simulink library "mobileRoboticsLib"  (R2022b)
settings: Solver=VariableStepAuto  StartTime=0.0  StopTime=10.0  RelTol=1e-3
undefined symbols (not defined in the file or in its folder): DiscIntNeverNeededParam, X, Y, Z
libraries: sm_lib x67, nesl_utility x25, $bdroot x12
(part 4 of 4)

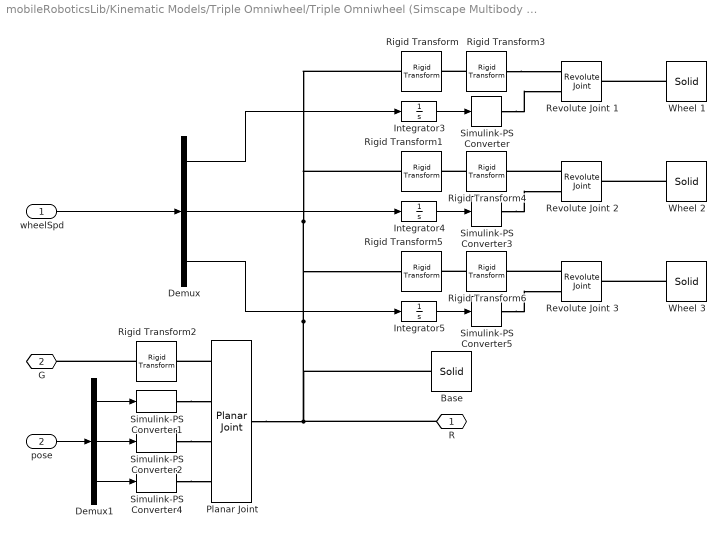
== system mobileRoboticsLib/Kinematic Models/Triple Omniwheel/Triple Omniwheel (Simscape Multibody Model) ==
  wheelSpd : Inport
  pose : Inport  Port=2
  Base : sm_lib/Body Elements/Solid  GraphicAmbientColor=[0.15 0.15 0.15 1.0]  BasedOnType=Mass  CenterOfMass=[0 0 0]  CenterOfMassUnits=m  GraphicDiffuseColor=chassisColor  CylinderLength=chassisThickness  CylinderLengthUnits=m  CylinderRadius=robotRadius-(wheelThickness/2)  CylinderRadiusUnits=m  Density=chassisMass  DensityUnits=kg/m^3  DoExposeReferenceFrame=on  GraphicEmissiveColor=[0.0 0.0 0.0 1.0]  ExportEntireGeometry=off  SerializedFrames=<Frames/>  MarkerShape=Sphere  MarkerSize=10  GraphicType=FromGeometry  InertiaType=CalculateFromGeometry  Mass=chassisMass  MassUnits=kg  MomentsOfInertia=[1 1 1]  MomentsOfInertiaUnits=kg*m^2  GraphicOpacity=1.0  ProductsOfInertia=[1 1 1]  ProductsOfInertiaUnits=kg*m^2  GraphicShininess=75  GraphicSpecularColor=[0.5 0.5 0.5 1.0]  GraphicVisPropType=SimpleVisualProperties  GeometryShape=Cylinder
  Demux : Demux  Outputs=3
  Demux1 : Demux  Outputs=3
  Integrator3 : Integrator
  Integrator4 : Integrator
  Integrator5 : Integrator
  Planar Joint : sm_lib/Joints/Planar Joint  JointMode=Normal  SenseConstraintForce=off  SenseConstraintForceX=off  SenseConstraintForceY=off  SenseConstraintForceZ=off  SenseConstraintTorque=off  SenseConstraintTorqueX=off  SenseConstraintTorqueY=off  SenseConstraintTorqueZ=off  SenseTotalForce=off  SenseTotalForceX=off  SenseTotalForceY=off  SenseTotalForceZ=off  SenseTotalTorque=off  SenseTotalTorqueX=off  SenseTotalTorqueY=off  SenseTotalTorqueZ=off  CompositeWrenchDir=FollowerOnBase  CompositeWrenchFrame=BaseFrame  PxEquilibriumPosition=0  PxEquilibriumPositionUnits=m  PxSpringStiffness=0  PxSpringStiffnessUnits=N/m  PxDampingCoefficient=0  PxDampingCoefficientUnits=N/(m/s)  PxTorqueActuationMode=ComputedTorque  PxMotionActuationMode=InputMotion  PxSensePosition=off  PxSenseVelocity=off  PxSenseAcceleration=off  PxSenseTorqueForce=off  PxSenseLowerLimitTorqueForce=off  PxSenseUpperLimitTorqueForce=off  PxLowerLimitSpecify=off  PxLowerLimitBound=-1  PxLowerLimitBoundUnits=m  PxLowerLimitStiffness=1e6  PxLowerLimitStiffnessUnits=N/m  PxLowerLimitDamping=1e3  PxLowerLimitDampingUnits=N/(m/s)  PxLowerLimitTransitionRegionWidth=1e-4  PxLowerLimitTransitionRegionWidthUnits=m  PxUpperLimitSpecify=off  PxUpperLimitBound=1  PxUpperLimitBoundUnits=m  PxUpperLimitStiffness=1e6  PxUpperLimitStiffnessUnits=N/m  PxUpperLimitDamping=1e3  PxUpperLimitDampingUnits=N/(m/s)  PxUpperLimitTransitionRegionWidth=1e-4  PxUpperLimitTransitionRegionWidthUnits=m  PxPositionTargetSpecify=on  PxPositionTargetPriority=High  PxPositionTargetValue=initX  PxPositionTargetValueUnits=m  PxVelocityTargetSpecify=off  PxVelocityTargetPriority=High  PxVelocityTargetValue=0  PxVelocityTargetValueUnits=m/s  PyEquilibriumPosition=0  PyEquilibriumPositionUnits=m  PySpringStiffness=0  PySpringStiffnessUnits=N/m  PyDampingCoefficient=0  PyDampingCoefficientUnits=N/(m/s)  PyTorqueActuationMode=ComputedTorque  PyMotionActuationMode=InputMotion  PySensePosition=off  PySenseVelocity=off  PySenseAcceleration=off  PySenseTorqueForce=off  PySenseLowerLimitTorqueForce=off  PySenseUpperLimitTorqueForce=off  PyLowerLimitSpecify=off  PyLowerLimitBound=-1  PyLowerLimitBoundUnits=m  PyLowerLimitStiffness=1e6  PyLowerLimitStiffnessUnits=N/m  PyLowerLimitDamping=1e3  PyLowerLimitDampingUnits=N/(m/s)  PyLowerLimitTransitionRegionWidth=1e-4  PyLowerLimitTransitionRegionWidthUnits=m  PyUpperLimitSpecify=off  PyUpperLimitBound=1  PyUpperLimitBoundUnits=m  PyUpperLimitStiffness=1e6  PyUpperLimitStiffnessUnits=N/m  PyUpperLimitDamping=1e3  PyUpperLimitDampingUnits=N/(m/s)  PyUpperLimitTransitionRegionWidth=1e-4  PyUpperLimitTransitionRegionWidthUnits=m  PyPositionTargetSpecify=on  PyPositionTargetPriority=High  PyPositionTargetValue=initY  PyPositionTargetValueUnits=m  PyVelocityTargetSpecify=off  PyVelocityTargetPriority=High  PyVelocityTargetValue=0  PyVelocityTargetValueUnits=m/s  RzEquilibriumPosition=0  RzEquilibriumPositionUnits=deg  RzSpringStiffness=0  RzSpringStiffnessUnits=N*m/deg  RzDampingCoefficient=0  RzDampingCoefficientUnits=N*m/(deg/s)  RzTorqueActuationMode=ComputedTorque  RzMotionActuationMode=InputMotion  RzSensePosition=off  RzSenseVelocity=off  RzSenseAcceleration=off  RzSenseTorqueForce=off  RzSenseLowerLimitTorqueForce=off  RzSenseUpperLimitTorqueForce=off  RzLowerLimitSpecify=off  RzLowerLimitBound=-90  RzLowerLimitBoundUnits=deg  RzLowerLimitStiffness=1e4  RzLowerLimitStiffnessUnits=N*m/deg  RzLowerLimitDamping=10  RzLowerLimitDampingUnits=N*m/(deg/s)  RzLowerLimitTransitionRegionWidth=0.1  RzLowerLimitTransitionRegionWidthUnits=deg  RzUpperLimitSpecify=off  RzUpperLimitBound=90  RzUpperLimitBoundUnits=deg  RzUpperLimitStiffness=1e4  RzUpperLimitStiffnessUnits=N*m/deg  RzUpperLimitDamping=10  RzUpperLimitDampingUnits=N*m/(deg/s)  RzUpperLimitTransitionRegionWidth=0.1  RzUpperLimitTransitionRegionWidthUnits=deg  RzPositionTargetSpecify=on  RzPositionTargetPriority=High  RzPositionTargetValue=initAngle  RzPositionTargetValueUnits=rad  RzVelocityTargetSpecify=off  RzVelocityTargetPriority=High  RzVelocityTargetValue=0  RzVelocityTargetValueUnits=deg/s
  Revolute Joint 1 : sm_lib/Joints/Revolute Joint  JointMode=Normal  SenseConstraintForce=off  SenseConstraintForceX=off  SenseConstraintForceY=off  SenseConstraintForceZ=off  SenseConstraintTorque=off  SenseConstraintTorqueX=off  SenseConstraintTorqueY=off  SenseConstraintTorqueZ=off  SenseTotalForce=off  SenseTotalForceX=off  SenseTotalForceY=off  SenseTotalForceZ=off  SenseTotalTorque=off  SenseTotalTorqueX=off  SenseTotalTorqueY=off  SenseTotalTorqueZ=off  CompositeWrenchDir=FollowerOnBase  CompositeWrenchFrame=BaseFrame  EquilibriumPosition=0  EquilibriumPositionUnits=deg  SpringStiffness=0  SpringStiffnessUnits=N*m/deg  DampingCoefficient=0  DampingCoefficientUnits=N*m/(deg/s)  TorqueActuationMode=ComputedTorque  MotionActuationMode=InputMotion  SensePosition=off  SenseVelocity=off  SenseAcceleration=off  SenseTorqueForce=off  SenseLowerLimitTorqueForce=off  SenseUpperLimitTorqueForce=off  LowerLimitSpecify=off  LowerLimitBound=-90  LowerLimitBoundUnits=deg  LowerLimitStiffness=1e4  LowerLimitStiffnessUnits=N*m/deg  LowerLimitDamping=10  LowerLimitDampingUnits=N*m/(deg/s)  LowerLimitTransitionRegionWidth=0.1  LowerLimitTransitionRegionWidthUnits=deg  UpperLimitSpecify=off  UpperLimitBound=90  UpperLimitBoundUnits=deg  UpperLimitStiffness=1e4  UpperLimitStiffnessUnits=N*m/deg  UpperLimitDamping=10  UpperLimitDampingUnits=N*m/(deg/s)  UpperLimitTransitionRegionWidth=0.1  UpperLimitTransitionRegionWidthUnits=deg  PositionTargetSpecify=off  PositionTargetPriority=High  PositionTargetValue=0  PositionTargetValueUnits=deg  VelocityTargetSpecify=off  VelocityTargetPriority=High  VelocityTargetValue=0  VelocityTargetValueUnits=deg/s
  Revolute Joint 2 : sm_lib/Joints/Revolute Joint  JointMode=Normal  SenseConstraintForce=off  SenseConstraintForceX=off  SenseConstraintForceY=off  SenseConstraintForceZ=off  SenseConstraintTorque=off  SenseConstraintTorqueX=off  SenseConstraintTorqueY=off  SenseConstraintTorqueZ=off  SenseTotalForce=off  SenseTotalForceX=off  SenseTotalForceY=off  SenseTotalForceZ=off  SenseTotalTorque=off  SenseTotalTorqueX=off  SenseTotalTorqueY=off  SenseTotalTorqueZ=off  CompositeWrenchDir=FollowerOnBase  CompositeWrenchFrame=BaseFrame  EquilibriumPosition=0  EquilibriumPositionUnits=deg  SpringStiffness=0  SpringStiffnessUnits=N*m/deg  DampingCoefficient=0  DampingCoefficientUnits=N*m/(deg/s)  TorqueActuationMode=ComputedTorque  MotionActuationMode=InputMotion  SensePosition=off  SenseVelocity=off  SenseAcceleration=off  SenseTorqueForce=off  SenseLowerLimitTorqueForce=off  SenseUpperLimitTorqueForce=off  LowerLimitSpecify=off  LowerLimitBound=-90  LowerLimitBoundUnits=deg  LowerLimitStiffness=1e4  LowerLimitStiffnessUnits=N*m/deg  LowerLimitDamping=10  LowerLimitDampingUnits=N*m/(deg/s)  LowerLimitTransitionRegionWidth=0.1  LowerLimitTransitionRegionWidthUnits=deg  UpperLimitSpecify=off  UpperLimitBound=90  UpperLimitBoundUnits=deg  UpperLimitStiffness=1e4  UpperLimitStiffnessUnits=N*m/deg  UpperLimitDamping=10  UpperLimitDampingUnits=N*m/(deg/s)  UpperLimitTransitionRegionWidth=0.1  UpperLimitTransitionRegionWidthUnits=deg  PositionTargetSpecify=off  PositionTargetPriority=High  PositionTargetValue=0  PositionTargetValueUnits=deg  VelocityTargetSpecify=off  VelocityTargetPriority=High  VelocityTargetValue=0  VelocityTargetValueUnits=deg/s
  Revolute Joint 3 : sm_lib/Joints/Revolute Joint  JointMode=Normal  SenseConstraintForce=off  SenseConstraintForceX=off  SenseConstraintForceY=off  SenseConstraintForceZ=off  SenseConstraintTorque=off  SenseConstraintTorqueX=off  SenseConstraintTorqueY=off  SenseConstraintTorqueZ=off  SenseTotalForce=off  SenseTotalForceX=off  SenseTotalForceY=off  SenseTotalForceZ=off  SenseTotalTorque=off  SenseTotalTorqueX=off  SenseTotalTorqueY=off  SenseTotalTorqueZ=off  CompositeWrenchDir=FollowerOnBase  CompositeWrenchFrame=BaseFrame  EquilibriumPosition=0  EquilibriumPositionUnits=deg  SpringStiffness=0  SpringStiffnessUnits=N*m/deg  DampingCoefficient=0  DampingCoefficientUnits=N*m/(deg/s)  TorqueActuationMode=ComputedTorque  MotionActuationMode=InputMotion  SensePosition=off  SenseVelocity=off  SenseAcceleration=off  SenseTorqueForce=off  SenseLowerLimitTorqueForce=off  SenseUpperLimitTorqueForce=off  LowerLimitSpecify=off  LowerLimitBound=-90  LowerLimitBoundUnits=deg  LowerLimitStiffness=1e4  LowerLimitStiffnessUnits=N*m/deg  LowerLimitDamping=10  LowerLimitDampingUnits=N*m/(deg/s)  LowerLimitTransitionRegionWidth=0.1  LowerLimitTransitionRegionWidthUnits=deg  UpperLimitSpecify=off  UpperLimitBound=90  UpperLimitBoundUnits=deg  UpperLimitStiffness=1e4  UpperLimitStiffnessUnits=N*m/deg  UpperLimitDamping=10  UpperLimitDampingUnits=N*m/(deg/s)  UpperLimitTransitionRegionWidth=0.1  UpperLimitTransitionRegionWidthUnits=deg  PositionTargetSpecify=off  PositionTargetPriority=High  PositionTargetValue=0  PositionTargetValueUnits=deg  VelocityTargetSpecify=off  VelocityTargetPriority=High  VelocityTargetValue=0  VelocityTargetValueUnits=deg/s
  Rigid Transform : sm_lib/Frames and Transforms/Rigid Transform  TranslationMethod=Cartesian  TranslationStandardOffset=0  TranslationLengthUnit=m  TranslationStandardAxis=+Y  TranslationCartesianOffset=[robotRadius*cos(wheelAngles(1)) robotRadius*sin(wheelAngles(1)) 0]  TranslationROffset=0  TranslationROffsetUnits=m  TranslationZOffset=0  TranslationZOffsetUnits=m  TranslationThetaOffset=0  TranslationThetaOffsetUnits=deg  RotationMethod=AlignedAxes  RotationAngleUnits=deg  RotationStandardAxis=+Z  RotationAngle=0.0  RotationArbitraryAxis=[0 0 1]  FollAlignAxisA=+Z  BaseAlignAxisA=+Y  FollAlignAxisB=+X  BaseAlignAxisB=+X  RotationSequenceAxes=FollowerAxes  RotationSequence=XYX  RotationSequenceAngles=[0 0 0]  RotationSequenceAnglesUnits=deg  RotationMatrix=[1 0 0; 0 1 0; 0 0 1]
  Rigid Transform1 : sm_lib/Frames and Transforms/Rigid Transform  TranslationMethod=Cartesian  TranslationStandardOffset=0  TranslationLengthUnit=m  TranslationStandardAxis=+Y  TranslationCartesianOffset=[robotRadius*cos(wheelAngles(2)) robotRadius*sin(wheelAngles(2)) 0]  TranslationROffset=0  TranslationROffsetUnits=m  TranslationZOffset=0  TranslationZOffsetUnits=m  TranslationThetaOffset=0  TranslationThetaOffsetUnits=deg  RotationMethod=AlignedAxes  RotationAngleUnits=deg  RotationStandardAxis=+Z  RotationAngle=0.0  RotationArbitraryAxis=[0 0 1]  FollAlignAxisA=+Z  BaseAlignAxisA=+Y  FollAlignAxisB=+X  BaseAlignAxisB=+X  RotationSequenceAxes=FollowerAxes  RotationSequence=XYX  RotationSequenceAngles=[0 0 0]  RotationSequenceAnglesUnits=deg  RotationMatrix=[1 0 0; 0 1 0; 0 0 1]
  Rigid Transform2 : sm_lib/Frames and Transforms/Rigid Transform  TranslationMethod=StandardAxis  TranslationStandardOffset=wheelRadius  TranslationLengthUnit=m  TranslationStandardAxis=+Z  TranslationCartesianOffset=[0 0 0]  TranslationROffset=0  TranslationROffsetUnits=m  TranslationZOffset=0  TranslationZOffsetUnits=m  TranslationThetaOffset=0  TranslationThetaOffsetUnits=deg  RotationMethod=None  RotationAngleUnits=deg  RotationStandardAxis=+Z  RotationAngle=0.0  RotationArbitraryAxis=[0 0 1]  FollAlignAxisA=+Z  BaseAlignAxisA=+Y  FollAlignAxisB=+X  BaseAlignAxisB=+X  RotationSequenceAxes=FollowerAxes  RotationSequence=XYX  RotationSequenceAngles=[0 0 0]  RotationSequenceAnglesUnits=deg  RotationMatrix=[1 0 0; 0 1 0; 0 0 1]
  Rigid Transform3 : sm_lib/Frames and Transforms/Rigid Transform  TranslationMethod=None  TranslationStandardOffset=0  TranslationLengthUnit=m  TranslationStandardAxis=+Z  TranslationCartesianOffset=[0 0 0]  TranslationROffset=0  TranslationROffsetUnits=m  TranslationZOffset=0  TranslationZOffsetUnits=m  TranslationThetaOffset=0  TranslationThetaOffsetUnits=deg  RotationMethod=StandardAxis  RotationAngleUnits=rad  RotationStandardAxis=+Y  RotationAngle=pi/2-wheelAngles(1)  RotationArbitraryAxis=[0 0 1]  FollAlignAxisA=+X  BaseAlignAxisA=+Y  FollAlignAxisB=+Y  BaseAlignAxisB=+Z  RotationSequenceAxes=FollowerAxes  RotationSequence=XYX  RotationSequenceAngles=[0 0 0]  RotationSequenceAnglesUnits=deg  RotationMatrix=[1 0 0; 0 1 0; 0 0 1]
  Rigid Transform4 : sm_lib/Frames and Transforms/Rigid Transform  TranslationMethod=None  TranslationStandardOffset=0  TranslationLengthUnit=m  TranslationStandardAxis=+Z  TranslationCartesianOffset=[0 0 0]  TranslationROffset=0  TranslationROffsetUnits=m  TranslationZOffset=0  TranslationZOffsetUnits=m  TranslationThetaOffset=0  TranslationThetaOffsetUnits=deg  RotationMethod=StandardAxis  RotationAngleUnits=rad  RotationStandardAxis=+Y  RotationAngle=pi/2-wheelAngles(2)  RotationArbitraryAxis=[0 0 1]  FollAlignAxisA=+X  BaseAlignAxisA=+Y  FollAlignAxisB=+Y  BaseAlignAxisB=+Z  RotationSequenceAxes=FollowerAxes  RotationSequence=XYX  RotationSequenceAngles=[0 0 0]  RotationSequenceAnglesUnits=deg  RotationMatrix=[1 0 0; 0 1 0; 0 0 1]
  Rigid Transform5 : sm_lib/Frames and Transforms/Rigid Transform  TranslationMethod=Cartesian  TranslationStandardOffset=0  TranslationLengthUnit=m  TranslationStandardAxis=+Y  TranslationCartesianOffset=[robotRadius*cos(wheelAngles(3)) robotRadius*sin(wheelAngles(3)) 0]  TranslationROffset=0  TranslationROffsetUnits=m  TranslationZOffset=0  TranslationZOffsetUnits=m  TranslationThetaOffset=0  TranslationThetaOffsetUnits=deg  RotationMethod=AlignedAxes  RotationAngleUnits=deg  RotationStandardAxis=+Z  RotationAngle=0.0  RotationArbitraryAxis=[0 0 1]  FollAlignAxisA=+Z  BaseAlignAxisA=+Y  FollAlignAxisB=+X  BaseAlignAxisB=+X  RotationSequenceAxes=FollowerAxes  RotationSequence=XYX  RotationSequenceAngles=[0 0 0]  RotationSequenceAnglesUnits=deg  RotationMatrix=[1 0 0; 0 1 0; 0 0 1]
  Rigid Transform6 : sm_lib/Frames and Transforms/Rigid Transform  TranslationMethod=None  TranslationStandardOffset=0  TranslationLengthUnit=m  TranslationStandardAxis=+Z  TranslationCartesianOffset=[0 0 0]  TranslationROffset=0  TranslationROffsetUnits=m  TranslationZOffset=0  TranslationZOffsetUnits=m  TranslationThetaOffset=0  TranslationThetaOffsetUnits=deg  RotationMethod=StandardAxis  RotationAngleUnits=rad  RotationStandardAxis=+Y  RotationAngle=pi/2-wheelAngles(3)  RotationArbitraryAxis=[0 0 1]  FollAlignAxisA=+X  BaseAlignAxisA=+Y  FollAlignAxisB=+Y  BaseAlignAxisB=+Z  RotationSequenceAxes=FollowerAxes  RotationSequence=XYX  RotationSequenceAngles=[0 0 0]  RotationSequenceAnglesUnits=deg  RotationMatrix=[1 0 0; 0 1 0; 0 0 1]
  Simulink-PS Converter{,1..5} (6 alike) : nesl_utility/Simulink-PS Converter  PhysicalDomain=network_engine_domain  SubClassName=ps_input  LeftPortType=input  RightPortType=output  PseudoPeriodic=off  Frequencies=[]  NoiseDistribution=none  NoiseParameters=[]  Unit=1  AffineConversion=off  FilteringAndDerivatives=filter  SimscapeFilterOrder=2  InputFilterTimeConstant=timeConstant  UdotUserProvided=0
  Wheel 1 : sm_lib/Body Elements/Solid  GraphicAmbientColor=[0.15 0.15 0.15 1.0]  BasedOnType=Mass  CenterOfMass=[0 0 0]  CenterOfMassUnits=m  GraphicDiffuseColor=wheelColor  CylinderLength=wheelThickness  CylinderLengthUnits=m  CylinderRadius=wheelRadius  CylinderRadiusUnits=m  Density=1000  DensityUnits=kg/m^3  DoExposeReferenceFrame=on  GraphicEmissiveColor=[0.0 0.0 0.0 1.0]  ExportEntireGeometry=off  SerializedFrames=<Frames/>  MarkerShape=Sphere  MarkerSize=10  GraphicType=FromGeometry  InertiaType=CalculateFromGeometry  Mass=wheelMass  MassUnits=kg  MomentsOfInertia=[1 1 1]  MomentsOfInertiaUnits=kg*m^2  GraphicOpacity=1.0  ProductsOfInertia=[1 1 1]  ProductsOfInertiaUnits=kg*m^2  GraphicShininess=75  GraphicSpecularColor=[0.5 0.5 0.5 1.0]  GraphicVisPropType=SimpleVisualProperties  GeometryShape=Cylinder
  Wheel 2 : sm_lib/Body Elements/Solid  GraphicAmbientColor=[0.15 0.15 0.15 1.0]  BasedOnType=Mass  CenterOfMass=[0 0 0]  CenterOfMassUnits=m  GraphicDiffuseColor=wheelColor  CylinderLength=wheelThickness  CylinderLengthUnits=m  CylinderRadius=wheelRadius  CylinderRadiusUnits=m  Density=1000  DensityUnits=kg/m^3  DoExposeReferenceFrame=on  GraphicEmissiveColor=[0.0 0.0 0.0 1.0]  ExportEntireGeometry=off  SerializedFrames=<Frames/>  MarkerShape=Sphere  MarkerSize=10  GraphicType=FromGeometry  InertiaType=CalculateFromGeometry  Mass=wheelMass  MassUnits=kg  MomentsOfInertia=[1 1 1]  MomentsOfInertiaUnits=kg*m^2  GraphicOpacity=1.0  ProductsOfInertia=[1 1 1]  ProductsOfInertiaUnits=kg*m^2  GraphicShininess=75  GraphicSpecularColor=[0.5 0.5 0.5 1.0]  GraphicVisPropType=SimpleVisualProperties  GeometryShape=Cylinder
  Wheel 3 : sm_lib/Body Elements/Solid  GraphicAmbientColor=[0.15 0.15 0.15 1.0]  BasedOnType=Mass  CenterOfMass=[0 0 0]  CenterOfMassUnits=m  GraphicDiffuseColor=wheelColor  CylinderLength=wheelThickness  CylinderLengthUnits=m  CylinderRadius=wheelRadius  CylinderRadiusUnits=m  Density=1000  DensityUnits=kg/m^3  DoExposeReferenceFrame=on  GraphicEmissiveColor=[0.0 0.0 0.0 1.0]  ExportEntireGeometry=off  SerializedFrames=<Frames/>  MarkerShape=Sphere  MarkerSize=10  GraphicType=FromGeometry  InertiaType=CalculateFromGeometry  Mass=wheelMass  MassUnits=kg  MomentsOfInertia=[1 1 1]  MomentsOfInertiaUnits=kg*m^2  GraphicOpacity=1.0  ProductsOfInertia=[1 1 1]  ProductsOfInertiaUnits=kg*m^2  GraphicShininess=75  GraphicSpecularColor=[0.5 0.5 0.5 1.0]  GraphicVisPropType=SimpleVisualProperties  GeometryShape=Cylinder
  R : PMIOPort  Side=Right
  G : PMIOPort  Port=2  Side=Right
  wires:
  wheelSpd/1 -> Demux/1
  Demux1/1 -> Simulink-PS Converter1/1
  Demux1/2 -> Simulink-PS Converter2/1
  Demux1/3 -> Simulink-PS Converter4/1
  pose/1 -> Demux1/1
  Integrator5/1 -> Simulink-PS Converter5/1
  Integrator3/1 -> Simulink-PS Converter/1
  Integrator4/1 -> Simulink-PS Converter3/1
  Demux/1 -> Integrator3/1
  Demux/2 -> Integrator4/1
  Demux/3 -> Integrator5/1
  connections:
  Simulink-PS Converter1/RConn1 -- Planar Joint/LConn2
  Rigid Transform2/LConn1 -- G/RConn1
  Simulink-PS Converter4/RConn1 -- Planar Joint/LConn4
  Simulink-PS Converter2/RConn1 -- Planar Joint/LConn3
  Planar Joint/LConn1 -- Rigid Transform2/RConn1
  R/RConn1 -- Planar Joint/RConn1 -- Base/RConn1 -- Rigid Transform/LConn1 -- Rigid Transform1/LConn1 -- Rigid Transform5/LConn1
  Rigid Transform6/LConn1 -- Rigid Transform5/RConn1
  Rigid Transform3/RConn1 -- Revolute Joint 1/LConn1
  Revolute Joint 3/LConn1 -- Rigid Transform6/RConn1
  Revolute Joint 2/LConn1 -- Rigid Transform4/RConn1
  Simulink-PS Converter3/RConn1 -- Revolute Joint 2/LConn2
  Simulink-PS Converter5/RConn1 -- Revolute Joint 3/LConn2
  Wheel 1/RConn1 -- Revolute Joint 1/RConn1
  Rigid Transform3/LConn1 -- Rigid Transform/RConn1
  Simulink-PS Converter/RConn1 -- Revolute Joint 1/LConn2
  Wheel 2/RConn1 -- Revolute Joint 2/RConn1
  Rigid Transform4/LConn1 -- Rigid Transform1/RConn1
  Wheel 3/RConn1 -- Revolute Joint 3/RConn1

== system mobileRoboticsLib/Kinematic Models/Triple Omniwheel/Triple Omniwheel Forward Kinematics ==
  wheelSpd : Inport
  MATLAB Function : MATLAB Function  TreatAsAtomicUnit=on
  bodySpd : Outport  VectorParamsAs1DForOutWhenUnconnected=off
  wires:
  wheelSpd/1 -> MATLAB Function/1(wheelSpeeds)  "wheelSpeeds"
  MATLAB Function/1(bodySpeed) -> bodySpd/1  "bodySpeed"

== system mobileRoboticsLib/Kinematic Models/Triple Omniwheel/Triple Omniwheel Inverse Kinematics  ==
  vRef : Inport
  MATLAB Function : MATLAB Function  TreatAsAtomicUnit=on
  wheelSpd : Outport  VectorParamsAs1DForOutWhenUnconnected=off
  wires:
  MATLAB Function/1(wheelSpeeds) -> wheelSpd/1  "wheelSpeeds"
  vRef/1 -> MATLAB Function/1(bodySpeed)  "bodySpeed"

== system mobileRoboticsLib/Kinematic Models/Triple Omniwheel/Triple Omniwheel Simulation ==
  wheelSpd : Inport
  Generic Robot Simulation : $bdroot/Utilities/Generic Vehicle Simulation  initX=initX  initY=initY  initAngle=initAngle  Ts=Ts
  Triple Omniwheel Forward Kinematics : $bdroot/Kinematic Models/Triple Omniwheel/Triple Omniwheel Forward Kinematics  wheelRadius=wheelRadius  robotRadius=robotRadius  wheelAngles=wheelAngles
  pose : Outport  VectorParamsAs1DForOutWhenUnconnected=off
  wires:
  wheelSpd/1 -> Triple Omniwheel Forward Kinematics/1
  Triple Omniwheel Forward Kinematics/1 -> Generic Robot Simulation/1
  Generic Robot Simulation/1 -> pose/1

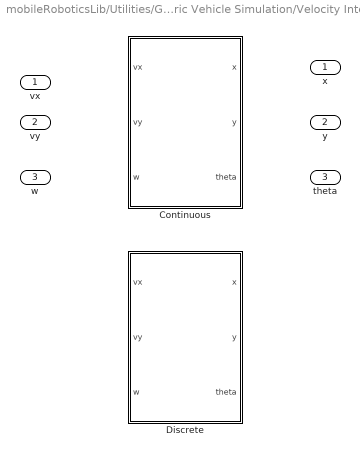
== system mobileRoboticsLib/Utilities/Generic Vehicle Simulation/Velocity Integrator ==
  "vx " : Inport
  "vy " : Inport  Port=2
  "w " : Inport  Port=3
  Continuous : Subsystem  VariantControl=mode==1
  Discrete : Subsystem  VariantControl=mode==2
  " x" : Outport  VectorParamsAs1DForOutWhenUnconnected=off
  " y" : Outport  Port=2  VectorParamsAs1DForOutWhenUnconnected=off
  " theta" : Outport  Port=3  VectorParamsAs1DForOutWhenUnconnected=off

== system mobileRoboticsLib/Kinematic Models/Four-Wheel Steering/Four-Wheel Steering Inverse Kinematics/Inverse Kinematics ==
  ref : Inport
  Front Steering : MATLAB Function  TreatAsAtomicUnit=on  VariantControl=mode==1
  Parallel Steering : MATLAB Function  TreatAsAtomicUnit=on  VariantControl=mode==2
  Zero Sideslip : MATLAB Function  TreatAsAtomicUnit=on  VariantControl=mode==3
  " wheelSpeeds" : Outport  VectorParamsAs1DForOutWhenUnconnected=off
  " steerAngles" : Outport  Port=2  VectorParamsAs1DForOutWhenUnconnected=off

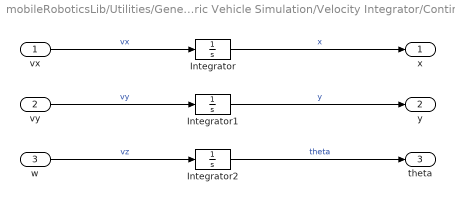
== system mobileRoboticsLib/Utilities/Generic Vehicle Simulation/Velocity Integrator/Continuous ==
  vx : Inport
  vy : Inport  Port=2
  w : Inport  Port=3
  Integrator : Integrator  InitialCondition=initX
  Integrator1 : Integrator  InitialCondition=initY
  Integrator2 : Integrator  InitialCondition=initAngle
  x : Outport  VectorParamsAs1DForOutWhenUnconnected=off
  y : Outport  Port=2  VectorParamsAs1DForOutWhenUnconnected=off
  theta : Outport  Port=3  VectorParamsAs1DForOutWhenUnconnected=off
  wires:
  Integrator1/1 -> y/1  "y"
  vy/1 -> Integrator1/1  "vy"
  Integrator/1 -> x/1  "x"
  vx/1 -> Integrator/1  "vx"
  w/1 -> Integrator2/1  "vz"
  Integrator2/1 -> theta/1  "theta"

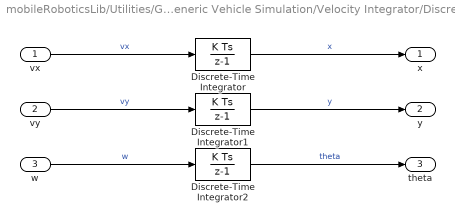
== system mobileRoboticsLib/Utilities/Generic Vehicle Simulation/Velocity Integrator/Discrete ==
  vx : Inport
  vy : Inport  Port=2
  w : Inport  Port=3
  Discrete-Time Integrator : DiscreteIntegrator  InitialCondition=initX  SampleTime=Ts  ICPrevOutput=DiscIntNeverNeededParam  ICPrevScaledInput=DiscIntNeverNeededParam
  Discrete-Time Integrator1 : DiscreteIntegrator  InitialCondition=initY  SampleTime=Ts  ICPrevOutput=DiscIntNeverNeededParam  ICPrevScaledInput=DiscIntNeverNeededParam
  Discrete-Time Integrator2 : DiscreteIntegrator  InitialCondition=initAngle  SampleTime=Ts  ICPrevOutput=DiscIntNeverNeededParam  ICPrevScaledInput=DiscIntNeverNeededParam
  x : Outport  VectorParamsAs1DForOutWhenUnconnected=off
  y : Outport  Port=2  VectorParamsAs1DForOutWhenUnconnected=off
  theta : Outport  Port=3  VectorParamsAs1DForOutWhenUnconnected=off
  wires:
  Discrete-Time Integrator2/1 -> theta/1  "theta"
  w/1 -> Discrete-Time Integrator2/1  "w"
  vx/1 -> Discrete-Time Integrator/1  "vx"
  Discrete-Time Integrator/1 -> x/1  "x"
  vy/1 -> Discrete-Time Integrator1/1  "vy"
  Discrete-Time Integrator1/1 -> y/1  "y"

== matlab function mobileRoboticsLib/Kinematic Models/Four-Wheel Mecanum/Four-Wheel Mecanum Forward Kinematics/MATLAB Function ==
  settings: updateMethod=DISCRETE
  data: wheelSpeeds input; bodySpeed output; wheelRadius parameter; wheelBase parameter; wheelTrack parameter
function bodySpeed = fourWheelMecanumFwdKin(wheelSpeeds,wheelRadius,wheelBase,wheelTrack)
    
    % Initialize FourWheelMecanum object
    persistent robot
    if isempty(robot)
        robot = FourWheelMecanum(wheelRadius,wheelBase,wheelTrack);
    end
    
    % Run object's forward kinematics method
    bodySpeed = forwardKinematics(robot,wheelSpeeds);

end

== matlab function mobileRoboticsLib/Kinematic Models/Four-Wheel Mecanum/Four-Wheel Mecanum Inverse Kinematics/MATLAB Function ==
  data: bodySpeed input; wheelRadius parameter; wheelSpeeds output; wheelBase parameter; wheelTrack parameter
function wheelSpeeds = fourWheelMecanumInvKin(bodySpeed,wheelRadius,wheelBase,wheelTrack)
    
    % Initialize FourWheelMecanum object
    persistent robot
    if isempty(robot)
        robot = FourWheelMecanum(wheelRadius,wheelBase,wheelTrack);
    end
    
    % Run object's inverse kinematics method
    wheelSpeeds = inverseKinematics(robot,bodySpeed);

end

== matlab function mobileRoboticsLib/Environments/Multi-Robot Environment/Visualize ==
  data: visuals input; poses input; waypts input; numRobots parameter; ranges input; objs input; objDetParams input; robotDetParams input; plotSensorLines parameter; showRobotIds parameter
function visualizeWaypointsAndObjects(visuals,poses,waypts,numRobots,ranges,objs, ...
                                      objDetParams,robotDetParams,plotSensorLines, showRobotIds)

    coder.extrinsic('internal.multiRobotVizWorld')
    internal.multiRobotVizWorld(numRobots,visuals,poses,waypts,ranges,objs, ... 
                                objDetParams,robotDetParams,showRobotIds,plotSensorLines);

end

== matlab function mobileRoboticsLib/Utilities/Assign to Maximum Size ==
  data: u input; y output size=maxLength; maxLength parameter
function y = assign2max(u,maxLength)

y = zeros(maxLength,1);
numElems = min(maxLength,size(u,1));
y(1:numElems) = u(1:numElems);

== matlab function mobileRoboticsLib/Kinematic Models/Generic Omniwheel/Generic Omniwheel Forward Kinematics/MATLAB Function ==
  settings: updateMethod=DISCRETE
  data: wheelSpeeds input; bodySpeed output; wheelRadius parameter; wheelPositions parameter; wheelAngles parameter
function bodySpeed = genericOmniFwdKin(wheelSpeeds,wheelRadius,wheelPositions,wheelAngles)
    
    % Initialize TripleOmniwheel object
    persistent robot
    if isempty(robot)
        robot = GenericOmniwheel(wheelRadius,wheelPositions,wheelAngles);
    end
    
    % Run object's forward kinematics method
    bodySpeed = forwardKinematics(robot,wheelSpeeds);

end

== matlab function mobileRoboticsLib/Kinematic Models/Generic Omniwheel/Generic Omniwheel Inverse Kinematics /MATLAB Function ==
  data: bodySpeed input; wheelRadius parameter; wheelPositions parameter; wheelSpeeds output; wheelAngles parameter
function wheelSpeeds = genericOmniInverseKinematics(bodySpeed,wheelRadius,wheelPositions,wheelAngles)
    
    % Initialize TripleOmniwheel object
    persistent robot
    if isempty(robot)
        robot = GenericOmniwheel(wheelRadius,wheelPositions,wheelAngles);
    end
    
    % Run object's inverse kinematics method
    wheelSpeeds = inverseKinematics(robot,bodySpeed);

end

== matlab function mobileRoboticsLib/Environments/Multi-Robot Visualizer/Assign to Maximum Size ==
  data: u input; y output size=maxLength; maxLength parameter
function y = assign2max(u,maxLength)

y = zeros(maxLength,1);
numElems = min(maxLength,size(u,1));
y(1:numElems) = u(1:numElems);

== matlab function mobileRoboticsLib/Environments/Multi-Robot Visualizer/Assign to Maximum Size1 ==
  data: u input; y output size=maxLength; maxLength parameter
function y = assign2max(u,maxLength)

y = zeros(maxLength,1);
numElems = min(maxLength,size(u,1));
y(1:numElems) = u(1:numElems);

== matlab function mobileRoboticsLib/Kinematic Models/Differential Drive/Differential Drive Forward Kinematics/MATLAB Function ==
  settings: updateMethod=DISCRETE
  data: wL input; v output; wR input; wheelRadius parameter; wheelBase parameter; w output
function [v,w] = diffDriveFwdKin(wL,wR,wheelRadius,wheelBase)
    
    % Initialize DifferentialDrive object
    persistent robot
    if isempty(robot)
        robot = DifferentialDrive(wheelRadius,wheelBase);
    end
    
    % Run object's forward kinematics method
    [v,w] = forwardKinematics(robot,wL,wR);

end

== matlab function mobileRoboticsLib/Kinematic Models/Differential Drive/Differential Drive Inverse Kinematics/MATLAB Function ==
  data: v input; wL output; w input; wR output; wheelRadius parameter; wheelBase parameter
function [wL,wR] = diffDriveInvKin(v,w,wheelRadius,wheelBase)
    
    % Initialize DifferentialDrive object
    persistent robot
    if isempty(robot)
        robot = DifferentialDrive(wheelRadius,wheelBase);
    end
    
    % Run object's forward kinematics method
    [wL,wR] = inverseKinematics(robot,v,w);

end

== matlab function mobileRoboticsLib/Kinematic Models/Four-Wheel Steering/Four-Wheel Steering Forward Kinematics/MATLAB Function ==
  settings: updateMethod=DISCRETE
  data: wheelSpeeds input; bodySpeed output; wheelRadius parameter; frontWheelDist parameter; rearWheelDist parameter; steerAngles input
function bodySpeed = fourWheelSteerFwdKin(wheelSpeeds,wheelRadius,frontWheelDist,rearWheelDist, steerAngles) ...
    
    % Initialize Four-Wheel Steering object
    persistent robot
    if isempty(robot)
        robot = FourWheelSteering(wheelRadius,[frontWheelDist,rearWheelDist]);
    end
    
    % Run object's forward kinematics method
    bodySpeed = forwardKinematics(robot,wheelSpeeds,steerAngles);

end

== matlab function mobileRoboticsLib/Kinematic Models/Triple Omniwheel/Triple Omniwheel Inverse Kinematics /MATLAB Function ==
  data: bodySpeed input; wheelRadius parameter; wheelSpeeds output size=3; wheelAngles parameter; robotRadius parameter
function wheelSpeeds = tripleOmniInverseKinematics(bodySpeed,wheelRadius,wheelAngles, robotRadius)
    
    % Initialize TripleOmniwheel object
    persistent robot
    if isempty(robot)
        robot = TripleOmniwheel(wheelRadius,robotRadius,wheelAngles);
    end
    
    % Run object's inverse kinematics method
    wheelSpeeds = inverseKinematics(robot,bodySpeed);

end

== matlab function mobileRoboticsLib/Kinematic Models/Four-Wheel Steering/Four-Wheel Steering Inverse Kinematics/Inverse Kinematics/Front Steering ==
  data: ref input; wheelRadius parameter; wheelSpeeds output; frontWheelDist parameter; rearWheelDist parameter; steerAngles output
function [wheelSpeeds,steerAngles] = fourWheelSteerInvKinFrontSteer ...
         (ref,wheelRadius,frontWheelDist,rearWheelDist)
    % ref = [vx;w]
    
    % Initialize FourWheelSteering object
    persistent robot
    if isempty(robot)
        robot = FourWheelSteering(wheelRadius,[frontWheelDist,rearWheelDist]);
    end
    
    % Run object's inverse kinematics method
    [wheelSpeeds,steerAngles] = ...
        inverseKinematicsFrontSteer(robot,ref(1),ref(2));

end

== matlab function mobileRoboticsLib/Kinematic Models/Triple Omniwheel/Triple Omniwheel Forward Kinematics/MATLAB Function ==
  settings: updateMethod=DISCRETE
  data: wheelSpeeds input; bodySpeed output; wheelRadius parameter; robotRadius parameter; wheelAngles parameter
function bodySpeed = tripleOmniFwdKin(wheelSpeeds,wheelRadius,robotRadius,wheelAngles)
    
    % Initialize TripleOmniwheel object
    persistent robot
    if isempty(robot)
        robot = TripleOmniwheel(wheelRadius,robotRadius,wheelAngles);
    end
    
    % Run object's forward kinematics method
    bodySpeed = forwardKinematics(robot,wheelSpeeds);

end

== matlab function mobileRoboticsLib/Kinematic Models/Four-Wheel Steering/Four-Wheel Steering Inverse Kinematics/Inverse Kinematics/Zero Sideslip ==
  data: ref input; wheelRadius parameter; wheelSpeeds output; frontWheelDist parameter; rearWheelDist parameter; steerAngles output
function [wheelSpeeds,steerAngles] = fourWheelSteerInvKinZeroSideslip ...
         (ref,wheelRadius,frontWheelDist,rearWheelDist)
    % ref = [vx;w]

    % Initialize FourWheelSteering object
    persistent robot
    if isempty(robot)
        robot = FourWheelSteering(wheelRadius,[frontWheelDist,rearWheelDist]);
    end
    
    % Run object's inverse kinematics method
    [wheelSpeeds,steerAngles] = ... 
        inverseKinematicsZeroSideslip(robot,ref(1),ref(2));

end

== matlab function mobileRoboticsLib/Kinematic Models/Four-Wheel Steering/Four-Wheel Steering Inverse Kinematics/Inverse Kinematics/Parallel Steering ==
  data: ref input; wheelRadius parameter; wheelSpeeds output; frontWheelDist parameter; rearWheelDist parameter; steerAngles output
function [wheelSpeeds,steerAngles] = fourWheelSteerInvKinParallelSteer ...
         (ref,wheelRadius,frontWheelDist,rearWheelDist)
    % ref = [vx;vy]
    
    % Initialize FourWheelSteering object
    persistent robot
    if isempty(robot)
        robot = FourWheelSteering(wheelRadius,[frontWheelDist,rearWheelDist]);
    end
    
    % Run object's inverse kinematics method
    [wheelSpeeds,steerAngles] = ... 
        inverseKinematicsParallelSteer(robot,ref(1),ref(2));

end
